simulink model "ukl_reg_dysk"  (R2023b)
settings: Solver=VariableStepAuto  StartTime=0.0  StopTime=200  FixedStep=tc  RelTol=1e-3
values from neighbouring files (symbols this model uses):
  h1 = round(0.1*Tmax,2)    [PA_Lab6.m]
  h2 = round(0.5*Tmax,2)    [PA_Lab6.m]
  h3 = round(Tmax,2)    [PA_Lab6.m]
libraries: cstblocks x10
settings Model: Creator=RafalG  LastModifiedBy=User
settings SolverCC: AlgebraicLoopSolver=TrustRegion
settings DataIOCC: SaveFormat=Array  SignalLoggingSaveFormat=ModelDataLogs  ReturnWorkspaceOutputs=off
settings OptimizationCC: ReuseModelBlockBuffer=off  ExpressionDepthLimit=2147483647  LifeSpan=inf
settings DebuggingCC: UnderspecifiedInitializationDetection=Classic  MergeDetectMultiDrivingBlocksExec=none  SolverPrmCheckMsg=warning  FcnCallInpInsideContextMsg=warning  UnconnectedInputMsg=warning  UnconnectedOutputMsg=warning  UnconnectedLineMsg=warning  StateNameClashWarn=warning  SFUnexpectedBacktrackingDiag=warning  SFNoUnconditionalDefaultTransitionDiag=warning  SFExecutionAtInitializationDiag=none  ArithmeticOperatorsInVariantConditions=warning
settings HardwareCC: ProdBitPerPointer=32  ProdBitPerSizeT=32  ProdBitPerPtrDiffT=32  ProdLargestAtomicFloat=None  ProdIntDivRoundTo=Undefined  ProdEndianess=Unspecified  ProdWordSize=32  ProdHWDeviceType=32-bit Generic
settings ModelReferenceCC: EnableRefExpFcnMdlSchedulingChecks=on  PropagateSignalLabelsOutOfModel=off
settings SFSimCC: SimUseLocalCustomCode=off  CustomCodeUndefinedFunction=UseInterfaceOnly
settings RTWCC: RTWUseLocalCustomCode=off
settings CodeAppCC: StateflowObjectComments=on
settings GRTTargetCC: TargetLangStandard=C89/C90 (ANSI)  CombineOutputUpdateFcns=off  GRTInterface=on
settings ConfigComp: CovMetricSettings=dw  CovSaveCumulativeToWorkspaceVar=on  CovSaveSingleToWorkspaceVar=on  CovExternalEMLEnable=off

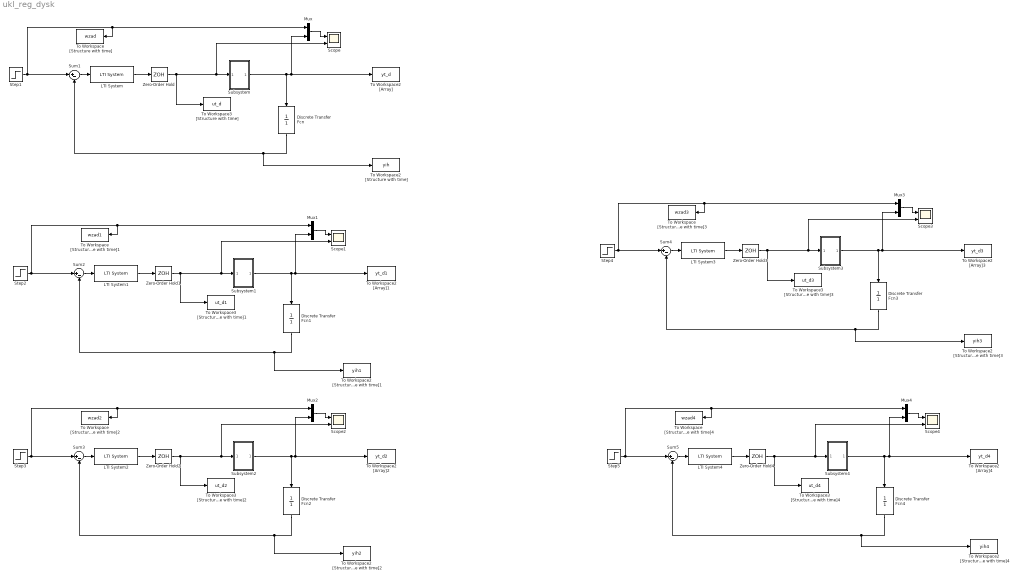
== system ukl_reg_dysk ==
  Discrete Transfer Fcn : DiscreteTransferFcn  Denominator=[1]  SampleTime=h1
  Discrete Transfer Fcn1 : DiscreteTransferFcn  Denominator=[1]  SampleTime=h2
  Discrete Transfer Fcn2 : DiscreteTransferFcn  Denominator=[1]  SampleTime=h3
  Discrete Transfer Fcn3 : DiscreteTransferFcn  Denominator=[1]  SampleTime=h1
  Discrete Transfer Fcn4 : DiscreteTransferFcn  Denominator=[1]  SampleTime=h1
  LTI System : cstblocks/LTI System  sys=Hr  IC=[]  PadeOrder=0
  LTI System1 : cstblocks/LTI System  sys=Hr2  IC=[]  PadeOrder=0
  LTI System2 : cstblocks/LTI System  sys=Hr3  IC=[]  PadeOrder=0
  LTI System3 : cstblocks/LTI System  sys=Hr4  IC=[]  PadeOrder=0
  LTI System4 : cstblocks/LTI System  sys=Hr5  IC=[]  PadeOrder=0
  Mux{,1..4} (5 alike) : Mux  Inputs=2
  Scope{,1..4} (5 alike) : Scope  NumInputPorts=2
  Step{1..5} (5 alike) : Step  Time=0  SampleTime=0
  Subsystem : Subsystem
  Subsystem1 : Subsystem
  Subsystem2 : Subsystem
  Subsystem3 : Subsystem
  Subsystem4 : Subsystem
  Sum{1..5} (5 alike) : Sum  Inputs=|+-
  To Workspace [Structure with time] : ToWorkspace  VariableName=wzad  SaveFormat=Structure With Time  SampleTime=h1
  To Workspace [Structure with time]1 : ToWorkspace  VariableName=wzad1  SaveFormat=Structure With Time  SampleTime=h2
  To Workspace [Structure with time]2 : ToWorkspace  VariableName=wzad2  SaveFormat=Structure With Time  SampleTime=h3
  To Workspace [Structure with time]3 : ToWorkspace  VariableName=wzad3  SaveFormat=Structure With Time  SampleTime=h1
  To Workspace [Structure with time]4 : ToWorkspace  VariableName=wzad4  SaveFormat=Structure With Time  SampleTime=h1
  To Workspace2 [Array] : ToWorkspace  VariableName=yt_d
  To Workspace2 [Array]1 : ToWorkspace  VariableName=yt_d1
  To Workspace2 [Array]2 : ToWorkspace  VariableName=yt_d2
  To Workspace2 [Array]3 : ToWorkspace  VariableName=yt_d3
  To Workspace2 [Array]4 : ToWorkspace  VariableName=yt_d4
  To Workspace2 [Structure with time] : ToWorkspace  VariableName=yih  SaveFormat=Structure With Time  SampleTime=h1
  To Workspace2 [Structure with time]1 : ToWorkspace  VariableName=yih1  SaveFormat=Structure With Time  SampleTime=h2
  To Workspace2 [Structure with time]2 : ToWorkspace  VariableName=yih2  SaveFormat=Structure With Time  SampleTime=h3
  To Workspace2 [Structure with time]3 : ToWorkspace  VariableName=yih3  SaveFormat=Structure With Time  SampleTime=h1
  To Workspace2 [Structure with time]4 : ToWorkspace  VariableName=yih4  SaveFormat=Structure With Time  SampleTime=h1
  To Workspace3 [Structure with time] : ToWorkspace  VariableName=ut_d  SaveFormat=Timeseries  SampleTime=h1
  To Workspace3 [Structure with time]1 : ToWorkspace  VariableName=ut_d1  SaveFormat=Timeseries  SampleTime=h2
  To Workspace3 [Structure with time]2 : ToWorkspace  VariableName=ut_d2  SaveFormat=Timeseries  SampleTime=h3
  To Workspace3 [Structure with time]3 : ToWorkspace  VariableName=ut_d3  SaveFormat=Timeseries  SampleTime=h1
  To Workspace3 [Structure with time]4 : ToWorkspace  VariableName=ut_d4  SaveFormat=Timeseries  SampleTime=h1
  Zero-Order Hold : ZeroOrderHold  SampleTime=h1
  Zero-Order Hold1 : ZeroOrderHold  SampleTime=h2
  Zero-Order Hold2 : ZeroOrderHold  SampleTime=h3
  Zero-Order Hold3 : ZeroOrderHold  SampleTime=h1
  Zero-Order Hold4 : ZeroOrderHold  SampleTime=h1
  wires:
  LTI System/1 -> Zero-Order Hold/1
  Sum1/1 -> LTI System/1
  Zero-Order Hold/1 -> To Workspace3 [Structure with time]/1, Subsystem/1(In1), Scope/2
  Subsystem/1(Out1) -> To Workspace2 [Array]/1, Mux/2, Discrete Transfer Fcn/1
  Mux/1 -> Scope/1
  Discrete Transfer Fcn/1 -> To Workspace2 [Structure with time]/1, Sum1/2
  Step1/1 -> Sum1/1, Mux/1, To Workspace [Structure with time]/1
  Step2/1 -> Sum2/1, Mux1/1, To Workspace [Structure with time]1/1
  Discrete Transfer Fcn1/1 -> To Workspace2 [Structure with time]1/1, Sum2/2
  Mux1/1 -> Scope1/1
  Zero-Order Hold1/1 -> To Workspace3 [Structure with time]1/1, Subsystem1/1(In1), Scope1/2
  Sum2/1 -> LTI System1/1
  Subsystem1/1(Out1) -> To Workspace2 [Array]1/1, Mux1/2, Discrete Transfer Fcn1/1
  LTI System1/1 -> Zero-Order Hold1/1
  Subsystem2/1(Out1) -> To Workspace2 [Array]2/1, Mux2/2, Discrete Transfer Fcn2/1
  LTI System2/1 -> Zero-Order Hold2/1
  Sum3/1 -> LTI System2/1
  Discrete Transfer Fcn2/1 -> To Workspace2 [Structure with time]2/1, Sum3/2
  Mux2/1 -> Scope2/1
  Step3/1 -> Sum3/1, Mux2/1, To Workspace [Structure with time]2/1
  Zero-Order Hold2/1 -> To Workspace3 [Structure with time]2/1, Subsystem2/1(In1), Scope2/2
  Mux3/1 -> Scope3/1
  LTI System3/1 -> Zero-Order Hold3/1
  Discrete Transfer Fcn3/1 -> To Workspace2 [Structure with time]3/1, Sum4/2
  Step4/1 -> Sum4/1, Mux3/1, To Workspace [Structure with time]3/1
  Subsystem3/1(Out1) -> To Workspace2 [Array]3/1, Mux3/2, Discrete Transfer Fcn3/1
  Zero-Order Hold3/1 -> To Workspace3 [Structure with time]3/1, Subsystem3/1(In1), Scope3/2
  Sum4/1 -> LTI System3/1
  Mux4/1 -> Scope4/1
  LTI System4/1 -> Zero-Order Hold4/1
  Discrete Transfer Fcn4/1 -> To Workspace2 [Structure with time]4/1, Sum5/2
  Step5/1 -> Sum5/1, Mux4/1, To Workspace [Structure with time]4/1
  Subsystem4/1(Out1) -> To Workspace2 [Array]4/1, Mux4/2, Discrete Transfer Fcn4/1
  Zero-Order Hold4/1 -> To Workspace3 [Structure with time]4/1, Subsystem4/1(In1), Scope4/2
  Sum5/1 -> LTI System4/1

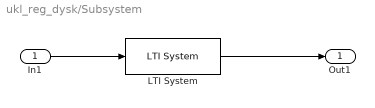
== system ukl_reg_dysk/Subsystem ==
  In1 : Inport
  LTI System : cstblocks/LTI System  sys=sys  IC=[]  PadeOrder=0
  Out1 : Outport
  wires:
  LTI System/1 -> Out1/1
  In1/1 -> LTI System/1

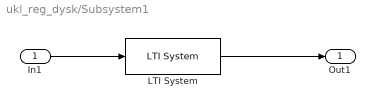
== system ukl_reg_dysk/Subsystem1 ==
  In1 : Inport
  LTI System : cstblocks/LTI System  sys=sys  IC=[]  PadeOrder=0
  Out1 : Outport
  wires:
  LTI System/1 -> Out1/1
  In1/1 -> LTI System/1

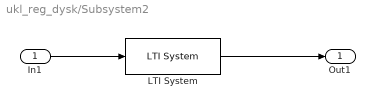
== system ukl_reg_dysk/Subsystem2 ==
  In1 : Inport
  LTI System : cstblocks/LTI System  sys=sys  IC=[]  PadeOrder=0
  Out1 : Outport
  wires:
  LTI System/1 -> Out1/1
  In1/1 -> LTI System/1

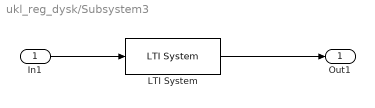
== system ukl_reg_dysk/Subsystem3 ==
  In1 : Inport
  LTI System : cstblocks/LTI System  sys=sys  IC=[]  PadeOrder=0
  Out1 : Outport
  wires:
  LTI System/1 -> Out1/1
  In1/1 -> LTI System/1

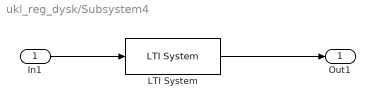
== system ukl_reg_dysk/Subsystem4 ==
  In1 : Inport
  LTI System : cstblocks/LTI System  sys=sys  IC=[]  PadeOrder=0
  Out1 : Outport
  wires:
  LTI System/1 -> Out1/1
  In1/1 -> LTI System/1
